simulink model "Open_loop_chopper_fed_MOSFET_separately_excited_DC_motor_drive"  (R2024a)
settings: Solver=VariableStepAuto  StartTime=0.0  StopTime=5  RelTol=1e-3
libraries: spsDCVoltageSourceLib x2, spsDCMachineLib x1, spsDiodeLib x1, spsMosfetLib x1, spsVoltageMeasurementLib x1, sps_lib x1
settings Model: Creator=kuria  LastModifiedBy=haris

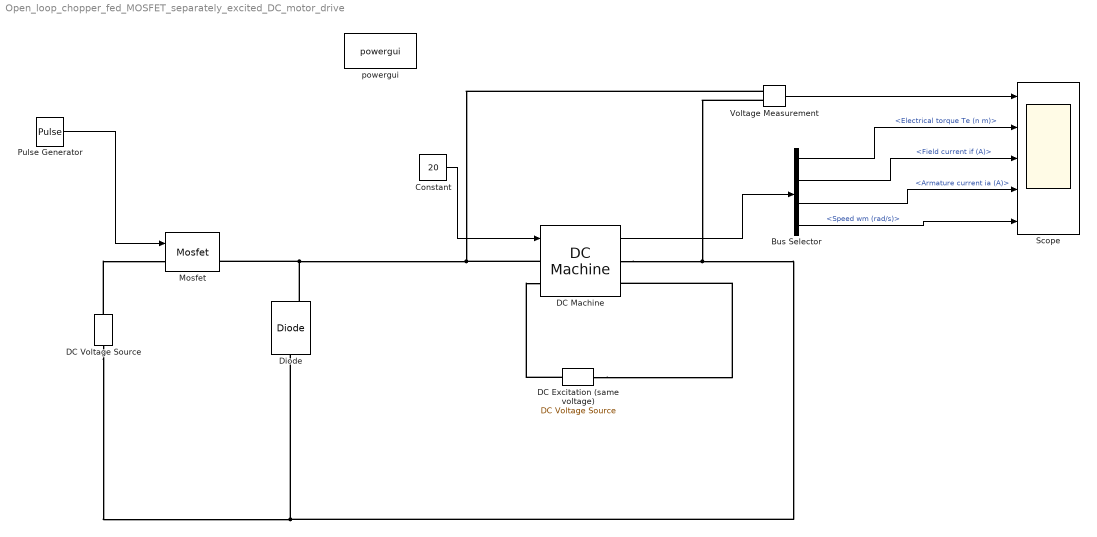
== system Open_loop_chopper_fed_MOSFET_separately_excited_DC_motor_drive ==
  Bus Selector : BusSelector  OutputSignals=Electrical torque Te (n m),Field current if (A),Armature current ia (A),Speed wm (rad/s)
  Constant : Constant  Value=20
  DC Excitation (same voltage) : spsDCVoltageSourceLib/DC Voltage Source  Amplitude=220  Measurements=None
  DC Machine : spsDCMachineLib/DC Machine  PresetModel=No  MechanicalLoad=Torque TL  FieldType=Wound  ShowDetailedParameters=on  MeasurementBus=off  RLa="[ 0.6  0.012]"  RLf="[ 240  120]"  Laf=1.8  MachineConstant=Torque constant (N.m/A)  Ke=1.8  Kt=1.8  J=1  Bm=0  Tf=0  w0=1  Ifinit=0.916666666666667  TsPowergui=0  TsBlock=-1
  DC Voltage Source : spsDCVoltageSourceLib/DC Voltage Source  Amplitude=220  Measurements=None
  Diode : spsDiodeLib/Diode  Ron=0.001  Lon=0  Vf=0.8  IC=0  UseSnubber=0  Rs=500  Cs=250e-9  Measurements=on
  Mosfet : spsMosfetLib/Mosfet  Ron=0.1  Lon=0  Rd=0.01  Vfd=0  IC=0  Rs=1e5  Cs=inf  Measurements=on
  Pulse Generator : DiscretePulseGenerator  PulseType=Time based  Period=0.02  PulseWidth=50
  Scope : Scope  NumInputPorts=5
  Voltage Measurement : spsVoltageMeasurementLib/Voltage Measurement  PhasorSimulation=off  OutputType=Complex  PSBequivalent=0
  powergui : sps_lib/powergui  Priority=1  SimulationMode=Continuous  SampleTime=50e-6  frequency=60  Iterations=50  frequencyindice=0  Pbase=100e6  ErrMax=1e-4  UnitsV=kV  UnitsW=MW  buscounter=0  FunctionMessages=off  echomessages=off  EnableUseOfTLC=off  CurrentSourceSwitches=off  DisableSnubberDevices=off  DisableRonSwitches=off  DisableVfSwitches=off  DisplayEquations=off  AutomaticDiscreteSolvers=off  SolverType=Tustin/Backward Euler (TBE)  Interpol=off  ExternalGateDelay=off  methode=off  Ts=100  x0status=blocks  SPID=on  SwTol=0  HookPort=off  NonlinearTolerance=1e-4  nMaxIteration=100  ContinueOnMaxIteration=off  RestoreLinks=warning  ResistiveCurrentMeasurement=off  Frange=[0:2:500]  Ylog=off  Xlog=on  ShowGrid=off  save=off  variable=ZData  structure=0  ZoomFFT=off  StartTime=0.0  cycles=1  DisplayStyle=1  fundamental=60  FreqAxis=off  MaxFrequency=1000  frequencyindicesteady=1  RmsSteady=1  display=off
  wires:
  Constant/1 -> DC Machine/1
  DC Machine/1 -> Bus Selector/1
  Bus Selector/1 -> Scope/2  "<Electrical torque Te (n m)>"
  Bus Selector/2 -> Scope/3  "<Field current if (A)>"
  Bus Selector/3 -> Scope/4  "<Armature current ia (A)>"
  Bus Selector/4 -> Scope/5  "<Speed wm (rad/s)>"
  Voltage Measurement/1 -> Scope/1
  Pulse Generator/1 -> Mosfet/1
  connections:
  DC Voltage Source/RConn1 -- Mosfet/LConn1
  DC Voltage Source/LConn1 -- Voltage Measurement/LConn2 -- DC Machine/RConn1 -- Diode/LConn1
  Diode/RConn1 -- DC Machine/LConn1 -- Voltage Measurement/LConn1 -- Mosfet/RConn1
  DC Excitation (same voltage)/LConn1 -- DC Machine/RConn2
  DC Excitation (same voltage)/RConn1 -- DC Machine/LConn2
